simulink model "Engine_Plant_SteadyState"  (R2026b)
settings: Solver=VariableStepAuto  StopTime=30
undefined symbols (not defined in the file): constants, delta_u_nom, ident, init, limits, p_a_nom, p_e_nom, simcfg, theta_a_nom, theta_m_nom, u_alpha_nom
settings Model: Creator=leont  LastModifiedBy=williamvandevoir

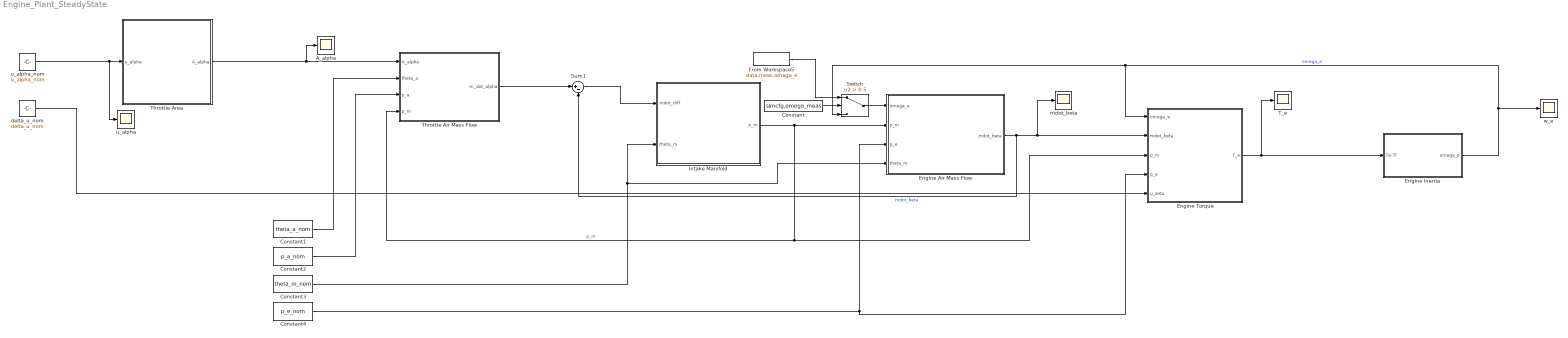
== system Engine_Plant_SteadyState ==
  A_alpha : Scope
      settings: DataLoggingVariableName=ScopeData4
  Constant : Constant  Value=simcfg.omega_meas
  Constant1 : Constant  Value=theta_a_nom
  Constant2 : Constant  Value=p_a_nom
  Constant3 : Constant  Value=theta_m_nom
  Constant4 : Constant  Value=p_e_nom
  Engine Air Mass Flow : Subsystem
  Engine Inertia : Subsystem
  Engine Torque : Subsystem
  From Workspace5 : FromWorkspace  VariableName=data.meas.omega_e
  Intake Manifold : Subsystem  Description=Adapted from Intake Manifold Exercise (pressure dynamics only): dp_m/dt = R*theta_m/Vm*(mdot_alpha - mdot_beta). One state; theta_m is an input; R instead of kappa*R.
  Sum1 : Sum  Inputs=|+-
  Switch : Switch  Criteria=u2 > Threshold  Threshold=0.5  SaturateOnIntegerOverflow=off  InputSameDT=off
  T_e : Scope
      settings: ActiveDisplayYMinimum=-24.090812904473726  ActiveDisplayYMaximum=17.370443961385767
  Throttle Air Mass Flow : Subsystem
  Throttle Area : Subsystem
  delta_u_nom : Constant  Value=delta_u_nom
  mdot_beta : Scope
      settings: ActiveDisplayYMinimum=0.0018042416431033796  ActiveDisplayYMaximum=0.0055634535738285336  DataLoggingVariableName=ScopeData2
  "u_alpha " : Scope
      settings: DataLoggingVariableName=ScopeData5
  u_alpha_nom : Constant  Value=u_alpha_nom
  w_e : Scope
      settings: ActiveDisplayYMinimum=119.00336194164404  ActiveDisplayYMaximum=158.56870514817743  DataLoggingVariableName=ScopeData3
  wires:
  Sum1/1 -> Intake Manifold/1(mdot_diff)
  Constant/1 -> Switch/2
  Throttle Air Mass Flow/1(m_dot_alpha) -> Sum1/1
  Engine Torque/1(T_e) -> Engine Inertia/1(Te-Tl), T_e/1
  Constant3/1 -> Intake Manifold/2(theta_m), Engine Air Mass Flow/4(theta_m)
  Throttle Area/1(A_alpha) -> A_alpha/1, Throttle Air Mass Flow/1(A_alpha)
  From Workspace5/1 -> Switch/1
  delta_u_nom/1 -> Engine Torque/5(u_zeta)
  Constant2/1 -> Throttle Air Mass Flow/3(p_a)
  Switch/1 -> Engine Air Mass Flow/1(omega_e)
  Intake Manifold/1(p_m) -> Engine Torque/3(p_m), Throttle Air Mass Flow/4(p_m), Engine Air Mass Flow/2(p_m)  "p_m"
  Engine Air Mass Flow/1(mdot_beta) -> Sum1/2, mdot_beta/1, Engine Torque/2(mdot_beta)  "mdot_beta"
  Constant1/1 -> Throttle Air Mass Flow/2(theta_a)
  Constant4/1 -> Engine Torque/4(p_e), Engine Air Mass Flow/3(p_e)
  Engine Inertia/1(omega_e) -> Switch/3, Engine Torque/1(omega_e), w_e/1  "omega_e"
  u_alpha_nom/1 -> "u_alpha "/1, Throttle Area/1(u_alpha)

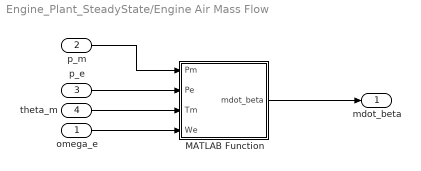
== system Engine_Plant_SteadyState/Engine Air Mass Flow ==
  omega_e : Inport
  p_m : Inport  Port=2
  p_e : Inport  Port=3
  theta_m : Inport  Port=4
  MATLAB Function : MATLAB Function  TreatAsAtomicUnit=on
  mdot_beta : Outport
  wires:
  p_e/1 -> MATLAB Function/2(Pe)
  theta_m/1 -> MATLAB Function/3(Tm)
  omega_e/1 -> MATLAB Function/4(We)
  MATLAB Function/1(mdot_beta) -> mdot_beta/1
  p_m/1 -> MATLAB Function/1(Pm)

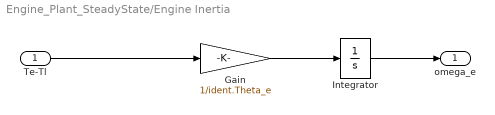
== system Engine_Plant_SteadyState/Engine Inertia ==
  Te-Tl : Inport
  Gain : Gain  Gain=1/ident.Theta_e
  Integrator : Integrator  InitialCondition=init.omega_e0  LimitOutput=on  UpperSaturationLimit=limits.w_max  LowerSaturationLimit=limits.w_min
  omega_e : Outport
  wires:
  Gain/1 -> Integrator/1
  Integrator/1 -> omega_e/1
  Te-Tl/1 -> Gain/1

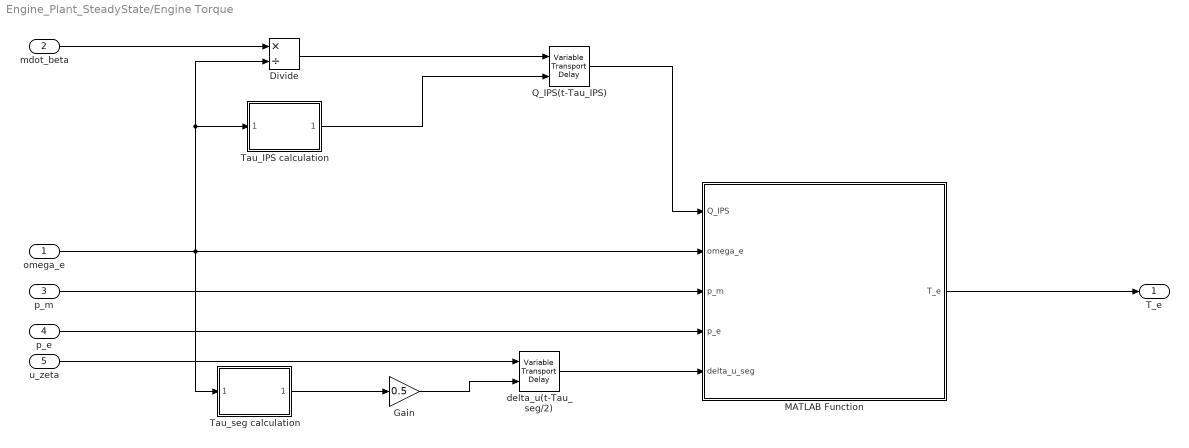
== system Engine_Plant_SteadyState/Engine Torque ==
  omega_e : Inport
  mdot_beta : Inport  Port=2
  p_m : Inport  Port=3
  p_e : Inport  Port=4
  u_zeta : Inport  Port=5
  Divide : Product  Inputs=*/
  Gain : Gain  Gain=0.5
  MATLAB Function : MATLAB Function  TreatAsAtomicUnit=on
  Q_IPS(t-Tau_IPS) : VariableTransportDelay  MaximumDelay=limits.tau_max  InitialOutput=init.q_init
  Tau_IPS calculation : MATLAB Function  TreatAsAtomicUnit=on
  Tau_seg calculation : MATLAB Function  TreatAsAtomicUnit=on
  delta_u(t-Tau_seg/2) : VariableTransportDelay  MaximumDelay=limits.tau_max  InitialOutput=init.du_init
  T_e : Outport
  wires:
  Gain/1 -> delta_u(t-Tau_seg/2)/2
  p_m/1 -> MATLAB Function/3(p_m)
  omega_e/1 -> Divide/2, Tau_IPS calculation/1(omega_e), Tau_seg calculation/1(omega_e), MATLAB Function/2(omega_e)
  Q_IPS(t-Tau_IPS)/1 -> MATLAB Function/1(Q_IPS)
  Tau_IPS calculation/1(Tau_IPS) -> Q_IPS(t-Tau_IPS)/2
  Tau_seg calculation/1(Tau_seg) -> Gain/1
  delta_u(t-Tau_seg/2)/1 -> MATLAB Function/5(delta_u_seg)
  u_zeta/1 -> delta_u(t-Tau_seg/2)/1
  MATLAB Function/1(T_e) -> T_e/1
  p_e/1 -> MATLAB Function/4(p_e)
  Divide/1 -> Q_IPS(t-Tau_IPS)/1
  mdot_beta/1 -> Divide/1

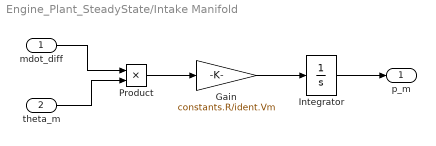
== system Engine_Plant_SteadyState/Intake Manifold ==
  mdot_diff : Inport
  theta_m : Inport  Port=2
  Gain : Gain  Gain=constants.R/ident.Vm
  Integrator : Integrator  InitialCondition=init.p_m0
  Product : Product
  p_m : Outport
  wires:
  mdot_diff/1 -> Product/1
  theta_m/1 -> Product/2
  Product/1 -> Gain/1
  Gain/1 -> Integrator/1
  Integrator/1 -> p_m/1

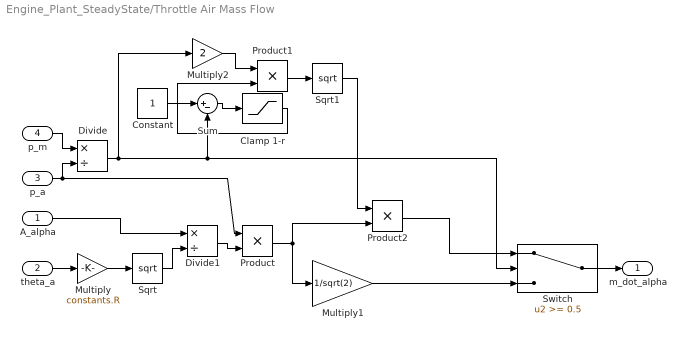
== system Engine_Plant_SteadyState/Throttle Air Mass Flow ==
  A_alpha : Inport
  theta_a : Inport  Port=2
  p_a : Inport  Port=3
  p_m : Inport  Port=4
  Clamp 1-r : Saturate  UpperLimit=inf  LowerLimit=0
  Constant : Constant
  Divide : Product  Inputs=*/
  Divide1 : Product  Inputs=*/
  Multiply : Gain  Gain=constants.R
  Multiply1 : Gain  Gain=1/sqrt(2)
  Multiply2 : Gain  Gain=2
  Product : Product
  Product1 : Product
  Product2 : Product
  Sqrt : Sqrt
  Sqrt1 : Sqrt
  Sum : Sum  Inputs=|+-
  Switch : Switch  Threshold=0.5  SaturateOnIntegerOverflow=off  InputSameDT=off
  m_dot_alpha : Outport
  wires:
  Multiply/1 -> Sqrt/1
  Multiply2/1 -> Product1/1
  Divide/1 -> Switch/2, Sum/2, Multiply2/1
  A_alpha/1 -> Divide1/1
  p_m/1 -> Divide/1
  Divide1/1 -> Product/2
  Product/1 -> Product2/2, Multiply1/1
  Constant/1 -> Sum/1
  Switch/1 -> m_dot_alpha/1
  theta_a/1 -> Multiply/1
  Multiply1/1 -> Switch/3
  Sqrt1/1 -> Product2/1
  Sqrt/1 -> Divide1/2
  Product1/1 -> Sqrt1/1
  p_a/1 -> Product/1, Divide/2
  Product2/1 -> Switch/1
  Sum/1 -> Clamp 1-r/1
  Clamp 1-r/1 -> Product1/2

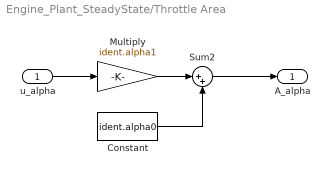
== system Engine_Plant_SteadyState/Throttle Area ==
  u_alpha : Inport
  Constant : Constant  Value=ident.alpha0
  Multiply : Gain  Gain=ident.alpha1
  Sum2 : Sum  Inputs=|++
  A_alpha : Outport
  wires:
  Multiply/1 -> Sum2/1
  Constant/1 -> Sum2/2
  u_alpha/1 -> Multiply/1
  Sum2/1 -> A_alpha/1

== matlab function Engine_Plant_SteadyState/Engine Torque/Tau_IPS calculation ==
  data: omega_e input; Tau_IPS output
function Tau_IPS = fcn(omega_e)

    if omega_e > 0
        Tau_IPS = 2*pi/omega_e;
    
    else
        Tau_IPS = 0;
    end

end

== matlab function Engine_Plant_SteadyState/Engine Torque/MATLAB Function ==
  data: Q_IPS input; omega_e input; p_m input; p_e input; delta_u_seg input; T_e output size=1; ident parameter; constants parameter
function T_e = fcn(Q_IPS, omega_e, p_m, p_e, delta_u_seg, ident, constants)

%% Parameters to identify: beta0, eta0, eta1

p_me0f = ident.beta0 * 4*pi/constants.Vd;
p_me0g = p_e - p_m;
e_zeta = 1 - constants.k_zeta*(delta_u_seg^2);
ep_mphi = (ident.eta0 + ident.eta1*omega_e)*e_zeta*constants.Hl*4*pi*Q_IPS/(constants.Vd*constants.lambda*constants.sigma0);

p_me = (ep_mphi - p_me0f - p_me0g);


T_e = p_me*constants.Vd/(4*pi);

== matlab function Engine_Plant_SteadyState/Engine Torque/Tau_seg calculation ==
  data: omega_e input; Tau_seg output
function Tau_seg = fcn(omega_e)

    if omega_e > 0
        Tau_seg = 4*pi/(5*omega_e);
    
    else
        Tau_seg = 0;
    end

end

== matlab function Engine_Plant_SteadyState/Engine Air Mass Flow/MATLAB Function ==
  data: Pm input; mdot_beta output size=1; Pe input; Tm input; We input; constants parameter; ident parameter
function mdot_beta = fcn(Pm, Pe, Tm, We, constants, ident)
% Engine Air Mass Flow: air mass flow leaving the intake manifold [kg/s]
% Inputs: Pm [Pa], Pe [Pa], Tm [K], We [rad/s]

% volumetric efficiency, pressure part (residual gas, polytropic expansion)
lam_lp = (constants.Vc + constants.Vd)/constants.Vd - (constants.Vc/constants.Vd) * (max(Pe/Pm, 0))^(1/constants.kappa);

% volumetric efficiency, speed part (linear in We, identified in milestone 2)
lam_lw = ident.gamma0 + ident.gamma1*We;

% air mass flow into the engine (four-stroke engine: factor 1/2)
mdot_e = 0.5 * Pm/(constants.R*Tm) * (lam_lp*lam_lw) * constants.Vd * We/(2*pi);

% air mass flow from the manifold (the rest is fuel, ratio lambda*sigma0)
mdot_beta = mdot_e / (1 + 1/(constants.lambda*constants.sigma0));
